simulink model "chaine_texte"  (R2023b)
settings: Solver=FixedStepDiscrete  StartTime=0.0  StopTime=Tsim  RelTol=1e-3
values from neighbouring files (symbols this model uses):
  dw = w    [partie4_q10.m]
  graine = 1    [extension_source_huffman.m]    (also in mes_parametres.m = mod(sum(c .* (1:numel(c)) * 31) + 7 * numel(c), 2^31 - 1); parametres_chaine.m = P.graine; parametres_perso.m = mod(sum(c .* (1:numel(c)) * 31) + 7 * numel(c), 2^31 - 1); partie4_q10.m = P.graine)
  sigma2v = N0 / 2    (= 0.0995267926384)    [partie5_q2.m]    (also in partie5_q3.m = N0 / 2; partie5_q4.m = N0 / 2; partie5_q5.m = Eb / e / 2)
  tabB1 = [0 0 1 1]    [partie5_q2.m]    (also in partie5_q3.m; partie5_q4.m; partie5_q5.m = M(m).tabB1)
  tabB2 = [0 1 0 1]    [partie5_q2.m]    (also in partie5_q3.m; partie5_q4.m; partie5_q5.m = M(m).tabB2)
  tabI = [ 1  1 -1 -1] / sqrt(2)    [partie5_q2.m]    (also in partie5_q3.m = [1 1 -1 -1] / sqrt(2); partie5_q4.m = [1 1 -1 -1] / sqrt(2); partie5_q5.m = M(m).tabI)
  tabQ = [ 1 -1  1 -1] / sqrt(2)    [partie5_q2.m]    (also in partie5_q3.m = [1 -1 1 -1] / sqrt(2); partie5_q4.m = [1 -1 1 -1] / sqrt(2); partie5_q5.m = M(m).tabQ)
  Tb = 1    [parametres.m]    (also in parametres_chaine.m; partie3_simulation.m; partie4_q10.m = 7; partie5_q2.m)
undefined symbols (not defined in the file or in its folder): tabIc, tabQc, Ts_c, Ts_nc
libraries: simulink x12
settings Model: Creator=e2604176  LastModifiedBy=e2604176
settings OptimizationCC: BooleanDataType=off

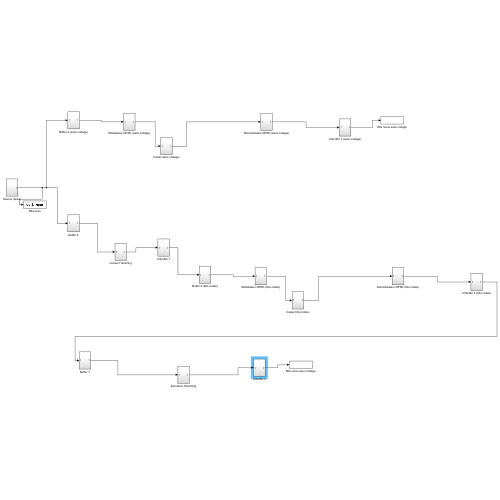
[thumbnail: Simulink's stored preview of the top-level diagram]
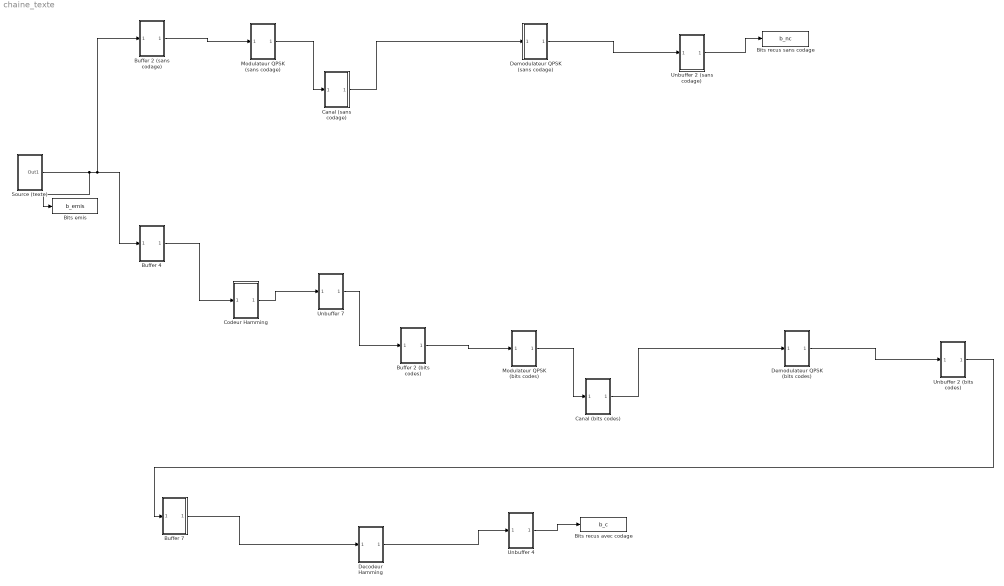
== system chaine_texte ==
  Bits emis : ToWorkspace  VariableName=b_emis  SampleTime=-1
  Bits recus avec codage : ToWorkspace  VariableName=b_c  SampleTime=-1
  Bits recus sans codage : ToWorkspace  VariableName=b_nc  SampleTime=-1
  Buffer 2 (bits codes) : Subsystem
  Buffer 2 (sans codage) : Subsystem
  Buffer 4 : Subsystem
  Buffer 7 : Subsystem
  Canal (bits codes) : Subsystem
  Canal (sans codage) : Subsystem
  Codeur Hamming : Subsystem
  Decodeur Hamming : Subsystem
  Demodulateur QPSK (bits codes) : Subsystem
  Demodulateur QPSK (sans codage) : Subsystem
  Modulateur QPSK (bits codes) : Subsystem
  Modulateur QPSK (sans codage) : Subsystem
  Source (texte) : Subsystem
  Unbuffer 2 (bits codes) : Subsystem
  Unbuffer 2 (sans codage) : Subsystem
  Unbuffer 4 : Subsystem
  Unbuffer 7 : Subsystem
  wires:
  Source (texte)/1(Out1) -> Buffer 4/1(In1), Buffer 2 (sans codage)/1(In1), Bits emis/1
  Buffer 2 (sans codage)/1(Out1) -> Modulateur QPSK (sans codage)/1(In1)
  Modulateur QPSK (sans codage)/1(Out1) -> Canal (sans codage)/1(In1)
  Canal (sans codage)/1(Out1) -> Demodulateur QPSK (sans codage)/1(In1)
  Demodulateur QPSK (sans codage)/1(Out1) -> Unbuffer 2 (sans codage)/1(In1)
  Unbuffer 2 (sans codage)/1(Out1) -> Bits recus sans codage/1
  Buffer 4/1(Out1) -> Codeur Hamming/1(In1)
  Codeur Hamming/1(Out1) -> Unbuffer 7/1(In1)
  Unbuffer 7/1(Out1) -> Buffer 2 (bits codes)/1(In1)
  Buffer 2 (bits codes)/1(Out1) -> Modulateur QPSK (bits codes)/1(In1)
  Modulateur QPSK (bits codes)/1(Out1) -> Canal (bits codes)/1(In1)
  Canal (bits codes)/1(Out1) -> Demodulateur QPSK (bits codes)/1(In1)
  Demodulateur QPSK (bits codes)/1(Out1) -> Unbuffer 2 (bits codes)/1(In1)
  Unbuffer 2 (bits codes)/1(Out1) -> Buffer 7/1(In1)
  Buffer 7/1(Out1) -> Decodeur Hamming/1(In1)
  Decodeur Hamming/1(Out1) -> Unbuffer 4/1(In1)
  Unbuffer 4/1(Out1) -> Bits recus avec codage/1

== system chaine_texte/Buffer 2 (bits codes) ==
  In1 : Inport
  C Buffer2 bloc : ZeroOrderHold  SampleTime=Ts_c
  C Buffer2 retards : simulink/Discrete/Tapped Delay  vinit=0  samptime=Tc  NumDelays=1  DelayOrder=Oldest  includeCurrent=on
  Out1 : Outport
  wires:
  C Buffer2 retards/1 -> C Buffer2 bloc/1
  C Buffer2 bloc/1 -> Out1/1
  In1/1 -> C Buffer2 retards/1

== system chaine_texte/Buffer 2 (sans codage) ==
  In1 : Inport
  NC Buffer2 bloc : ZeroOrderHold  SampleTime=Ts_nc
  NC Buffer2 retards : simulink/Discrete/Tapped Delay  vinit=0  samptime=Tb  NumDelays=1  DelayOrder=Oldest  includeCurrent=on
  Out1 : Outport
  wires:
  NC Buffer2 retards/1 -> NC Buffer2 bloc/1
  NC Buffer2 bloc/1 -> Out1/1
  In1/1 -> NC Buffer2 retards/1

== system chaine_texte/Buffer 4 ==
  In1 : Inport
  Buffer4 bloc : ZeroOrderHold  SampleTime=4*Tb
  Buffer4 retards : simulink/Discrete/Tapped Delay  vinit=0  samptime=Tb  NumDelays=3  DelayOrder=Oldest  includeCurrent=on
  Out1 : Outport
  wires:
  Buffer4 retards/1 -> Buffer4 bloc/1
  In1/1 -> Buffer4 retards/1
  Buffer4 bloc/1 -> Out1/1

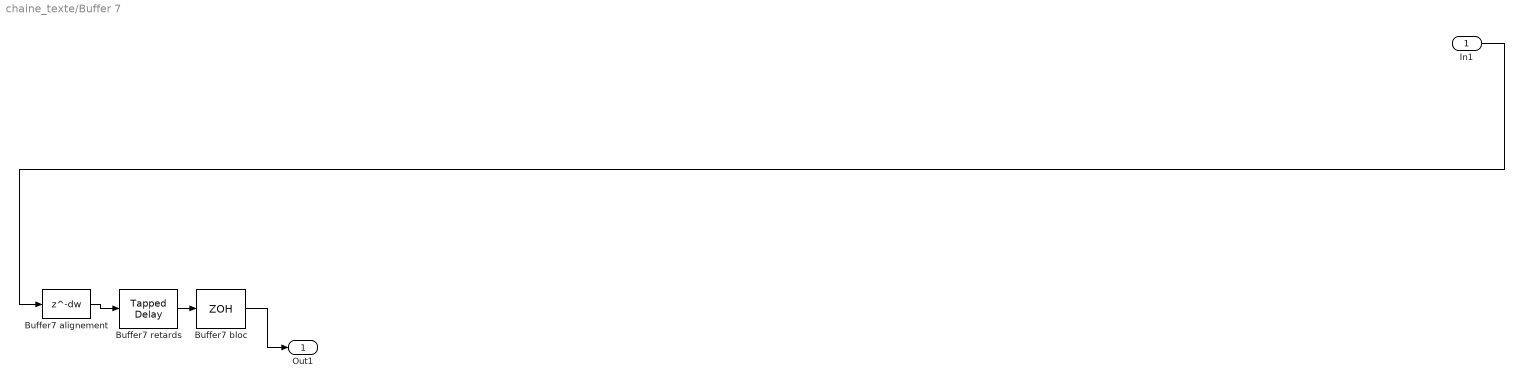
== system chaine_texte/Buffer 7 ==
  In1 : Inport
  Buffer7 alignement : Delay  DelayLength=dw
  Buffer7 bloc : ZeroOrderHold  SampleTime=4*Tb
  Buffer7 retards : simulink/Discrete/Tapped Delay  vinit=0  samptime=Tc  NumDelays=6  DelayOrder=Oldest  includeCurrent=on
  Out1 : Outport
  wires:
  Buffer7 alignement/1 -> Buffer7 retards/1
  Buffer7 bloc/1 -> Out1/1
  Buffer7 retards/1 -> Buffer7 bloc/1
  In1/1 -> Buffer7 alignement/1

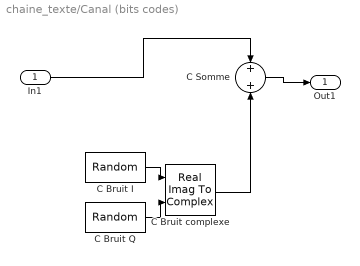
== system chaine_texte/Canal (bits codes) ==
  In1 : Inport
  C Bruit I : RandomNumber  Variance=sigma2v  Seed=graine + 3  SampleTime=Ts_c
  C Bruit Q : RandomNumber  Variance=sigma2v  Seed=graine + 3 + 1  SampleTime=Ts_c
  C Bruit complexe : RealImagToComplex
  C Somme : Sum
  Out1 : Outport
  wires:
  C Bruit complexe/1 -> C Somme/2
  C Bruit Q/1 -> C Bruit complexe/2
  C Somme/1 -> Out1/1
  C Bruit I/1 -> C Bruit complexe/1
  In1/1 -> C Somme/1

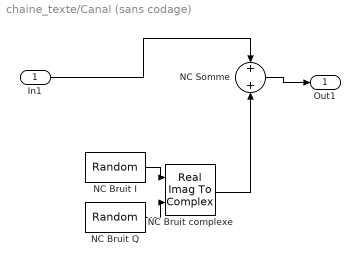
== system chaine_texte/Canal (sans codage) ==
  In1 : Inport
  NC Bruit I : RandomNumber  Variance=sigma2v  Seed=graine + 1  SampleTime=Ts_nc
  NC Bruit Q : RandomNumber  Variance=sigma2v  Seed=graine + 1 + 1  SampleTime=Ts_nc
  NC Bruit complexe : RealImagToComplex
  NC Somme : Sum
  Out1 : Outport
  wires:
  NC Bruit I/1 -> NC Bruit complexe/1
  NC Bruit complexe/1 -> NC Somme/2
  In1/1 -> NC Somme/1
  NC Bruit Q/1 -> NC Bruit complexe/2
  NC Somme/1 -> Out1/1

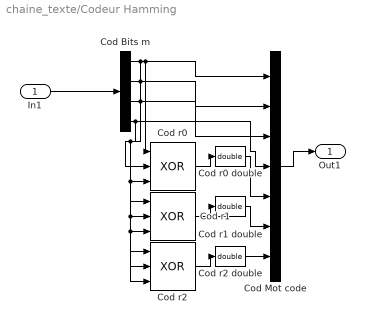
== system chaine_texte/Codeur Hamming ==
  In1 : Inport
  Cod Bits m : Demux
  Cod Mot code : Mux  Inputs=7
  Cod r0 : Logic  Operator=XOR  Inputs=3  AllPortsSameDT=off  OutDataTypeStr=boolean
  Cod r0 double : DataTypeConversion  OutDataTypeStr=double  SaturateOnIntegerOverflow=off  RndMeth=Floor
  Cod r1 : Logic  Operator=XOR  Inputs=3  AllPortsSameDT=off  OutDataTypeStr=boolean
  Cod r1 double : DataTypeConversion  OutDataTypeStr=double  SaturateOnIntegerOverflow=off  RndMeth=Floor
  Cod r2 : Logic  Operator=XOR  Inputs=3  AllPortsSameDT=off  OutDataTypeStr=boolean
  Cod r2 double : DataTypeConversion  OutDataTypeStr=double  SaturateOnIntegerOverflow=off  RndMeth=Floor
  Out1 : Outport
  wires:
  Cod r0 double/1 -> Cod Mot code/5
  Cod Bits m/2 -> Cod r1/2, Cod r2/1, Cod Mot code/2
  Cod Bits m/1 -> Cod r0/1, Cod Mot code/1, Cod r1/1
  Cod r1/1 -> Cod r1 double/1
  Cod r0/1 -> Cod r0 double/1
  Cod Bits m/3 -> Cod r1/3, Cod r2/2, Cod r0/2, Cod Mot code/3
  Cod Bits m/4 -> Cod r0/3, Cod r2/3, Cod Mot code/4
  Cod r1 double/1 -> Cod Mot code/6
  Cod r2/1 -> Cod r2 double/1
  Cod r2 double/1 -> Cod Mot code/7
  In1/1 -> Cod Bits m/1
  Cod Mot code/1 -> Out1/1

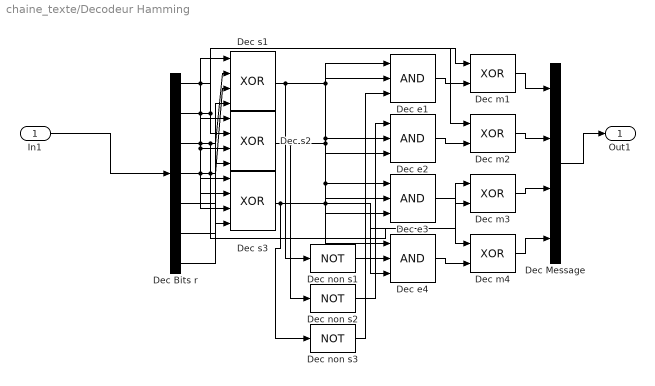
== system chaine_texte/Decodeur Hamming ==
  In1 : Inport
  Dec Bits r : Demux  Outputs=7
  Dec Message : Mux
  Dec e{1..4} (4 alike) : Logic  Inputs=3  AllPortsSameDT=off  OutDataTypeStr=boolean
  Dec m{1..4} (4 alike) : Logic  Operator=XOR  AllPortsSameDT=off  OutDataTypeStr=boolean
  Dec non s1 : Logic  Operator=NOT  Inputs=1  AllPortsSameDT=off  OutDataTypeStr=boolean
  Dec non s2 : Logic  Operator=NOT  Inputs=1  AllPortsSameDT=off  OutDataTypeStr=boolean
  Dec non s3 : Logic  Operator=NOT  Inputs=1  AllPortsSameDT=off  OutDataTypeStr=boolean
  Dec s1 : Logic  Operator=XOR  Inputs=4  AllPortsSameDT=off  OutDataTypeStr=boolean
  Dec s2 : Logic  Operator=XOR  Inputs=4  AllPortsSameDT=off  OutDataTypeStr=boolean
  Dec s3 : Logic  Operator=XOR  Inputs=4  AllPortsSameDT=off  OutDataTypeStr=boolean
  Out1 : Outport
  wires:
  Dec e1/1 -> Dec m1/2
  Dec e2/1 -> Dec m2/2
  Dec s3/1 -> Dec e2/3, Dec e3/3, Dec e4/3, Dec non s3/1
  Dec m1/1 -> Dec Message/1
  Dec Bits r/7 -> Dec s3/4
  Dec non s1/1 -> Dec e2/1
  Dec e4/1 -> Dec m4/2
  Dec m2/1 -> Dec Message/2
  Dec Bits r/2 -> Dec s2/2, Dec m2/1, Dec s3/1
  Dec s2/1 -> Dec e1/2, Dec e2/2, Dec e3/2, Dec non s2/1
  Dec Bits r/3 -> Dec s2/3, Dec s3/2, Dec s1/2, Dec m3/1
  Dec e3/1 -> Dec m3/2
  Dec Bits r/1 -> Dec s1/1, Dec s2/1, Dec m1/1
  Dec s1/1 -> Dec e3/1, Dec e4/1, Dec e1/1, Dec non s1/1
  Dec m3/1 -> Dec Message/3
  Dec non s2/1 -> Dec e4/2
  Dec Bits r/4 -> Dec s1/3, Dec m4/1, Dec s3/3
  Dec m4/1 -> Dec Message/4
  In1/1 -> Dec Bits r/1
  Dec Bits r/5 -> Dec s1/4
  Dec non s3/1 -> Dec e1/3
  Dec Bits r/6 -> Dec s2/4
  Dec Message/1 -> Out1/1

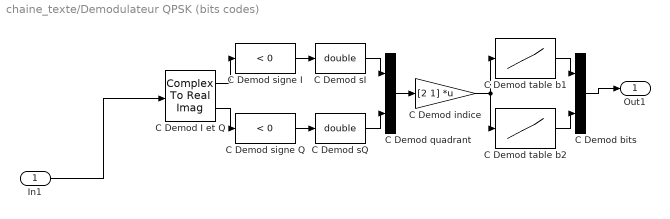
== system chaine_texte/Demodulateur QPSK (bits codes) ==
  In1 : Inport
  C Demod I et Q : ComplexToRealImag
  C Demod bits : Mux  Inputs=2
  C Demod indice : Gain  Gain=[2 1]  Multiplication=Matrix(K*u)
  C Demod quadrant : Mux  Inputs=2
  C Demod sI : DataTypeConversion  OutDataTypeStr=double  SaturateOnIntegerOverflow=off  RndMeth=Floor
  C Demod sQ : DataTypeConversion  OutDataTypeStr=double  SaturateOnIntegerOverflow=off  RndMeth=Floor
  C Demod signe I : simulink/Logic and Bit Operations/Compare To Constant  relop=<  const=0  OutDataTypeStr=boolean
  C Demod signe Q : simulink/Logic and Bit Operations/Compare To Constant  relop=<  const=0  OutDataTypeStr=boolean
  C Demod table b1 : Lookup_n-D  NumberOfTableDimensions=1  BreakpointsForDimension1=0:3  Table=tabB1  InternalRulePriority=Speed  RndMeth=Simplest
  C Demod table b2 : Lookup_n-D  NumberOfTableDimensions=1  BreakpointsForDimension1=0:3  Table=tabB2  InternalRulePriority=Speed  RndMeth=Simplest
  Out1 : Outport
  wires:
  C Demod I et Q/1 -> C Demod signe I/1
  C Demod sI/1 -> C Demod quadrant/1
  C Demod table b2/1 -> C Demod bits/2
  C Demod signe I/1 -> C Demod sI/1
  C Demod I et Q/2 -> C Demod signe Q/1
  C Demod indice/1 -> C Demod table b1/1, C Demod table b2/1
  C Demod signe Q/1 -> C Demod sQ/1
  C Demod table b1/1 -> C Demod bits/1
  C Demod sQ/1 -> C Demod quadrant/2
  C Demod quadrant/1 -> C Demod indice/1
  C Demod bits/1 -> Out1/1
  In1/1 -> C Demod I et Q/1

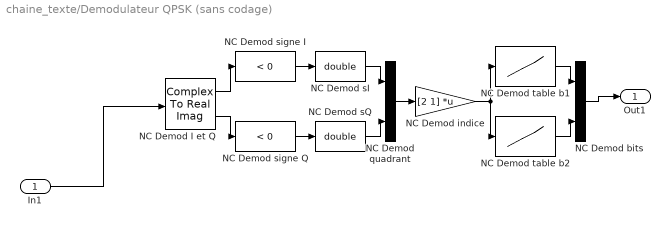
== system chaine_texte/Demodulateur QPSK (sans codage) ==
  In1 : Inport
  NC Demod I et Q : ComplexToRealImag
  NC Demod bits : Mux  Inputs=2
  NC Demod indice : Gain  Gain=[2 1]  Multiplication=Matrix(K*u)
  NC Demod quadrant : Mux  Inputs=2
  NC Demod sI : DataTypeConversion  OutDataTypeStr=double  SaturateOnIntegerOverflow=off  RndMeth=Floor
  NC Demod sQ : DataTypeConversion  OutDataTypeStr=double  SaturateOnIntegerOverflow=off  RndMeth=Floor
  NC Demod signe I : simulink/Logic and Bit Operations/Compare To Constant  relop=<  const=0  OutDataTypeStr=boolean
  NC Demod signe Q : simulink/Logic and Bit Operations/Compare To Constant  relop=<  const=0  OutDataTypeStr=boolean
  NC Demod table b1 : Lookup_n-D  NumberOfTableDimensions=1  BreakpointsForDimension1=0:3  Table=tabB1  InternalRulePriority=Speed  RndMeth=Simplest
  NC Demod table b2 : Lookup_n-D  NumberOfTableDimensions=1  BreakpointsForDimension1=0:3  Table=tabB2  InternalRulePriority=Speed  RndMeth=Simplest
  Out1 : Outport
  wires:
  NC Demod sI/1 -> NC Demod quadrant/1
  NC Demod I et Q/1 -> NC Demod signe I/1
  NC Demod quadrant/1 -> NC Demod indice/1
  NC Demod signe Q/1 -> NC Demod sQ/1
  NC Demod sQ/1 -> NC Demod quadrant/2
  NC Demod I et Q/2 -> NC Demod signe Q/1
  NC Demod signe I/1 -> NC Demod sI/1
  NC Demod indice/1 -> NC Demod table b1/1, NC Demod table b2/1
  NC Demod table b1/1 -> NC Demod bits/1
  NC Demod table b2/1 -> NC Demod bits/2
  In1/1 -> NC Demod I et Q/1
  NC Demod bits/1 -> Out1/1

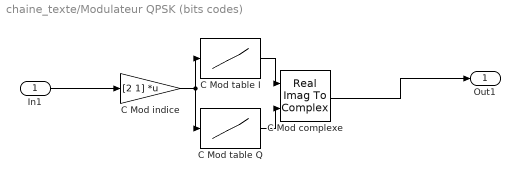
== system chaine_texte/Modulateur QPSK (bits codes) ==
  In1 : Inport
  C Mod complexe : RealImagToComplex
  C Mod indice : Gain  Gain=[2 1]  Multiplication=Matrix(K*u)
  C Mod table I : Lookup_n-D  NumberOfTableDimensions=1  BreakpointsForDimension1=0:3  Table=tabIc  InternalRulePriority=Speed  RndMeth=Simplest
  C Mod table Q : Lookup_n-D  NumberOfTableDimensions=1  BreakpointsForDimension1=0:3  Table=tabQc  InternalRulePriority=Speed  RndMeth=Simplest
  Out1 : Outport
  wires:
  In1/1 -> C Mod indice/1
  C Mod indice/1 -> C Mod table I/1, C Mod table Q/1
  C Mod table I/1 -> C Mod complexe/1
  C Mod table Q/1 -> C Mod complexe/2
  C Mod complexe/1 -> Out1/1

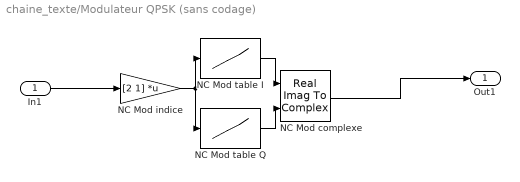
== system chaine_texte/Modulateur QPSK (sans codage) ==
  In1 : Inport
  NC Mod complexe : RealImagToComplex
  NC Mod indice : Gain  Gain=[2 1]  Multiplication=Matrix(K*u)
  NC Mod table I : Lookup_n-D  NumberOfTableDimensions=1  BreakpointsForDimension1=0:3  Table=tabI  InternalRulePriority=Speed  RndMeth=Simplest
  NC Mod table Q : Lookup_n-D  NumberOfTableDimensions=1  BreakpointsForDimension1=0:3  Table=tabQ  InternalRulePriority=Speed  RndMeth=Simplest
  Out1 : Outport
  wires:
  NC Mod complexe/1 -> Out1/1
  NC Mod indice/1 -> NC Mod table I/1, NC Mod table Q/1
  NC Mod table Q/1 -> NC Mod complexe/2
  NC Mod table I/1 -> NC Mod complexe/1
  In1/1 -> NC Mod indice/1

== system chaine_texte/Source (texte) ==
  Bit double : DataTypeConversion  OutDataTypeStr=double  SaturateOnIntegerOverflow=off  RndMeth=Floor
  Bits du texte : FromWorkspace  VariableName=entree  SampleTime=Tb  Interpolate=off  OutputAfterFinalValue=Setting to zero
  Out1 : Outport
  wires:
  Bits du texte/1 -> Bit double/1
  Bit double/1 -> Out1/1

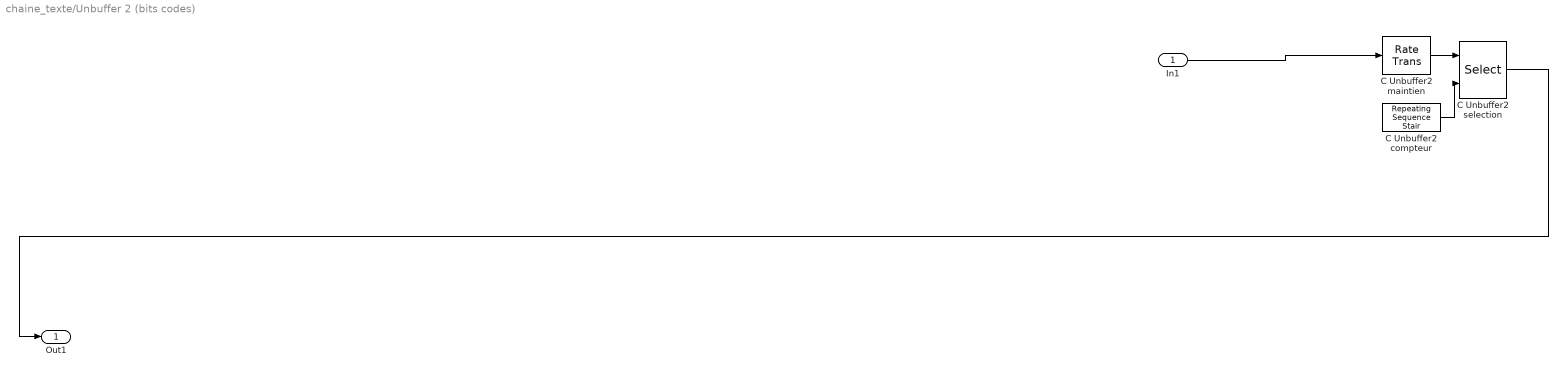
== system chaine_texte/Unbuffer 2 (bits codes) ==
  In1 : Inport
  C Unbuffer2 compteur : simulink/Sources/Repeating Sequence Stair  OutValues=1:2  tsamp=Tc  OutMin=[]  OutMax=[]  OutDataTypeStr=double  OutputDataTypeScalingMode=double  OutDataType=fixdt(0,8)  ConRadixGroup=Best Precision: Vector-wise  OutScaling=2^-12
  C Unbuffer2 maintien : RateTransition  OutPortSampleTime=Tc
  C Unbuffer2 selection : Selector  InputPortWidth=2  IndexOptions=Index vector (port)  Indices=[1 3]  OutputSizes=1
  Out1 : Outport
  wires:
  C Unbuffer2 compteur/1 -> C Unbuffer2 selection/2
  C Unbuffer2 maintien/1 -> C Unbuffer2 selection/1
  In1/1 -> C Unbuffer2 maintien/1
  C Unbuffer2 selection/1 -> Out1/1

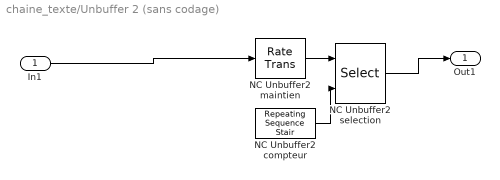
== system chaine_texte/Unbuffer 2 (sans codage) ==
  In1 : Inport
  NC Unbuffer2 compteur : simulink/Sources/Repeating Sequence Stair  OutValues=1:2  tsamp=Tb  OutMin=[]  OutMax=[]  OutDataTypeStr=double  OutputDataTypeScalingMode=double  OutDataType=fixdt(0,8)  ConRadixGroup=Best Precision: Vector-wise  OutScaling=2^-12
  NC Unbuffer2 maintien : RateTransition  OutPortSampleTime=Tb
  NC Unbuffer2 selection : Selector  InputPortWidth=2  IndexOptions=Index vector (port)  Indices=[1 3]  OutputSizes=1
  Out1 : Outport
  wires:
  NC Unbuffer2 maintien/1 -> NC Unbuffer2 selection/1
  NC Unbuffer2 selection/1 -> Out1/1
  NC Unbuffer2 compteur/1 -> NC Unbuffer2 selection/2
  In1/1 -> NC Unbuffer2 maintien/1

== system chaine_texte/Unbuffer 4 ==
  In1 : Inport
  Unbuffer4 compteur : simulink/Sources/Repeating Sequence Stair  OutValues=1:4  tsamp=Tb  OutMin=[]  OutMax=[]  OutDataTypeStr=double  OutputDataTypeScalingMode=double  OutDataType=fixdt(0,8)  ConRadixGroup=Best Precision: Vector-wise  OutScaling=2^-12
  Unbuffer4 maintien : RateTransition  OutPortSampleTime=Tb
  Unbuffer4 selection : Selector  InputPortWidth=4  IndexOptions=Index vector (port)  Indices=[1 3]  OutputSizes=1
  Out1 : Outport
  wires:
  Unbuffer4 maintien/1 -> Unbuffer4 selection/1
  Unbuffer4 compteur/1 -> Unbuffer4 selection/2
  Unbuffer4 selection/1 -> Out1/1
  In1/1 -> Unbuffer4 maintien/1

== system chaine_texte/Unbuffer 7 ==
  In1 : Inport
  Unbuffer7 compteur : simulink/Sources/Repeating Sequence Stair  OutValues=1:7  tsamp=Tc  OutMin=[]  OutMax=[]  OutDataTypeStr=double  OutputDataTypeScalingMode=double  OutDataType=fixdt(0,8)  ConRadixGroup=Best Precision: Vector-wise  OutScaling=2^-12
  Unbuffer7 maintien : RateTransition  OutPortSampleTime=Tc
  Unbuffer7 selection : Selector  InputPortWidth=7  IndexOptions=Index vector (port)  Indices=[1 3]  OutputSizes=1
  Out1 : Outport
  wires:
  Unbuffer7 compteur/1 -> Unbuffer7 selection/2
  In1/1 -> Unbuffer7 maintien/1
  Unbuffer7 selection/1 -> Out1/1
  Unbuffer7 maintien/1 -> Unbuffer7 selection/1
